simulink model "HybridShip0730"  (R2017b)
settings: Solver=ode3  StartTime=0.0  StopTime=10000  FixedStep=0.01  RelTol=1e-3
values from neighbouring files (symbols this model uses):
  Bat_Cap_Ah = Bat_Cap_kWh*1000/V_bus_nom    (= 930)    [ship_parameters0616.m]    (also in ship_parameters0616_utf8.m)
  Bat_R_int = 0.02    [ship_parameters0616.m]    (also in ship_parameters0616_utf8.m)
  Bat_SOC_init = 0.6    [ship_parameters0616.m]    (also in ship_parameters0616_utf8.m)
  C_bus = 20    [ship_parameters0616.m]    (also in ship_parameters0616_utf8.m)
  Elec_Eff = 0.92    [ship_parameters0616.m]    (also in ship_parameters0616_utf8.m)
  EMS_P_Hotel = 100    [ship_parameters0616.m]    (also in ship_parameters0616_utf8.m)
  F_env_const = 0    [ship_parameters0616.m]    (also in ship_parameters0616_utf8.m)
  Gear_Eff = 0.96    [ship_parameters0616.m]    (also in ship_parameters0616_utf8.m)
  Gear_Ratio = 6.08    [ship_parameters0616.m]    (also in ship_parameters0616_utf8.m)
  Gen_Fric_B = 0.1    [ship_parameters0616.m]    (also in ship_parameters0616_utf8.m)
  Gen_J = 50    [ship_parameters0616.m]    (also in ship_parameters0616_utf8.m)
  Gen_P_max = 500    [ship_parameters0616.m]    (also in ship_parameters0616_utf8.m)
  Gen_PI_I = 20    [ship_parameters0616.m]    (also in ship_parameters0616_utf8.m)
  Gen_PI_P = 50    [ship_parameters0616.m]    (also in ship_parameters0616_utf8.m)
  Gen_RPM_max = 1700    [ship_parameters0616.m]    (also in ship_parameters0616_utf8.m)
  Gen_RPM_nom = 1500    [ship_parameters0616.m]    (also in ship_parameters0616_utf8.m)
  Hull_K_R = P_effective_design_W / V_design_mps^3    (= 2651.6780136)    [ship_parameters0616.m]    (also in ship_parameters0616_utf8.m)
  K_Fv = (F_bollard - F_eff_design) / V_A_design^2    (= 1835.07128969)    [ship_parameters0616.m]    (also in ship_parameters0616_utf8.m)
  K_Fw = F_bollard / omega_prop_nom^2    (= 100.917597758)    [ship_parameters0616.m]    (also in ship_parameters0616_utf8.m)
  K_Qv = (Q_bollard - Q_prop_nom) / V_A_design^2    (= 212.582578785)    [ship_parameters0616.m]    (also in ship_parameters0616_utf8.m)
  K_Qw = Q_bollard / omega_prop_nom^2    (= 23.3814602154)    [ship_parameters0616.m]    (also in ship_parameters0616_utf8.m)
  Mot_PI_I = 5    [ship_parameters0616.m]    (also in ship_parameters0616_utf8.m)
  Mot_PI_P = 20    [ship_parameters0616.m]    (also in ship_parameters0616_utf8.m)
  Mot_T_max = (Mot_P_nom*1000)/(2*pi*Mot_RPM_nom/60)    (= 2228.16920329)    [ship_parameters0616.m]    (also in ship_parameters0616_utf8.m)
  Prop_J = 800    [ship_parameters0616.m]    (also in ship_parameters0616_utf8.m)
  R_tie = 0.002    [ship_parameters0616.m]    (also in ship_parameters0616_utf8.m)
  River_Current_mps = -1.0    (= -1)    [ship_parameters0616.m]    (also in ship_parameters0616_utf8.m)
  Shaft_B = 0    [ship_parameters0616.m]    (also in ship_parameters0616_utf8.m)
  Ship_Mass = 1.0e6    (= 1000000)    [ship_parameters0616.m]    (also in ship_parameters0616_utf8.m)
  V_bus_nom = 576    [ship_parameters0616.m]    (also in ship_parameters0616_utf8.m)
  wake_fraction = 0.15    [ship_parameters0616.m]    (also in ship_parameters0616_utf8.m)
libraries: simulink x6, simulink_extras x1
settings Model: Creator=Tommy  LastModifiedBy=Tommy

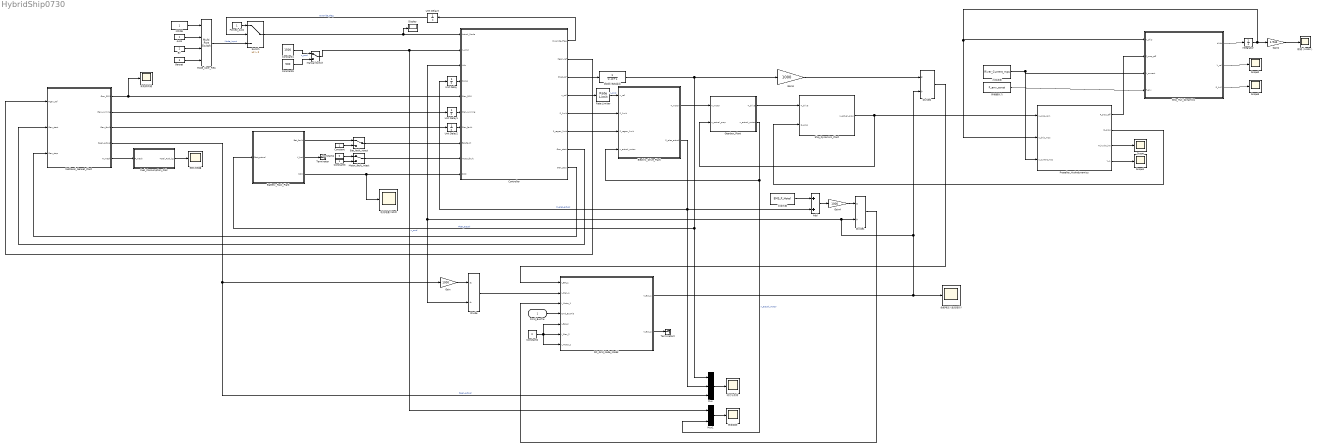
== system HybridShip0730 ==
  Cmd_BusTie : Inport
  Add : Sum
  Auto : Constant
  Bat_fault_Inject : ManualSwitch
  Battery_Pack_Plant : Subsystem
  Constant : Constant
  Constant1 : Constant  Value=1500  VectorParams1D=off  SampleTime=-1
  Constant2 : Constant  Value=0
  Constant3 : Constant
  Constant4 : Constant  Value=0
  Constant5 : Constant  Value=500  VectorParams1D=off  SampleTime=-1
  Controller : MATLAB Function  TreatAsAtomicUnit=on
  DCDC 响应延迟 : TransferFcn  Denominator=[0.1 1]
  DC_Grid_Node_Model : Subsystem
  Display : Display
  Divide : Product  Inputs=*/
  Divide1 : Product  Inputs=*/
  Divide2 : Product  Inputs=*/
  EV : Constant  Value=2
  Electric_Drive_Plant : Subsystem
  Forced_Auto : Constant
  Fuel_Consumption_Calc : Subsystem
  Gain : Gain  Gain=1000
  Gain2 : Gain  Gain=1.944
  Gain3 : Gain  Gain=1000
  Gain4 : Gain  Gain=1000
  Gearbox_Plant : Subsystem
  Genset : Constant  Value=3
  Integrator : Integrator
  MODE : Constant
  Manual Switch : ManualSwitch
  Methanol_Genset_Plant : Subsystem
  Mode_User_Req : MultiPortSwitch
  Motor_fault_Inject : ManualSwitch
  Mux : Mux  Inputs=3
  Mux1 : Mux  Inputs=2
  Propeller_Hydrodynamics : MATLAB Function  TreatAsAtomicUnit=on
  Rate Limiter : RateLimiter  RisingSlewLimit=50  FallingSlewLimit=-50  SampleTimeMode=inherited
  Scope{,1..3} (4 alike) : Scope
  Ship_Dynamics_Plant : Subsystem
  Ship_Hull_Dynamics : MATLAB Function  TreatAsAtomicUnit=on
  Switch : Switch  Criteria=u2 > Threshold
  Terminator : Terminator
  Terminator2 : Terminator
  Unit Delay{,1..3} (4 alike) : UnitDelay  SampleTime=0.1
  全船电压 (直流母排) : Scope
  动力与负荷 : Scope
  发电机转速 : Scope
  日用负载 : Constant  Value=EMS_P_Hotel
  河流流速 : Constant  Value=River_Current_mps
  燃料消耗量 : Scope
  环境额外力 : Constant  Value=F_env_const
  电池电量 (SOC) : Scope
  船速（knots） : Scope
  转速追踪 : Scope
  wires:
  Cmd_BusTie/1 -> DC_Grid_Node_Model/4(Cmd_BusTie)
  Methanol_Genset_Plant/4(Pgen_actual) -> Mux/3, Gain/1  "Pgen_actual"
  Gain/1 -> Divide/1
  Divide/1 -> DC_Grid_Node_Model/2(I_Gen_1)
  Controller/3(Pbat_ref) -> DCDC 响应延迟/1
  DCDC 响应延迟/1 -> Mux/1, Battery_Pack_Plant/1(Pbat_actual), Gain3/1  "Pbat_actual"
  Gain3/1 -> Divide2/1
  Divide2/1 -> DC_Grid_Node_Model/1(I_Bat_1)
  Electric_Drive_Plant/2(P_elec_actual) -> Add/2, Unit Delay/1, Mux/2  "P_elec_actual"
  Gain4/1 -> Divide1/1
  Divide1/1 -> DC_Grid_Node_Model/3(I_Motor_1)
  DC_Grid_Node_Model/1(V_Bus_1) -> Divide2/2, Divide/2, Controller/3(Vdc), Divide1/2, 全船电压 (直流母排)/1
  Methanol_Genset_Plant/2(Gen_running) -> Unit Delay1/1
  Battery_Pack_Plant/3(SOC) -> 电池电量 (SOC)/1, Controller/10(SOC)
  Controller/2(Pgen_ref) -> Methanol_Genset_Plant/1(Pgen_ref)
  Controller/7(Gen_start) -> Methanol_Genset_Plant/2(Gen_start)
  Controller/8(Gen_stop) -> Methanol_Genset_Plant/3(Gen_stop)
  Battery_Pack_Plant/2(V_bat) -> Terminator/1
  Battery_Pack_Plant/1(Bat_fault) -> Bat_fault_Inject/1
  DC_Grid_Node_Model/2(V_Bus_2) -> Terminator2/1
  Constant2/1 -> DC_Grid_Node_Model/7(I_Motor_2), DC_Grid_Node_Model/5(I_Bat_2), DC_Grid_Node_Model/6(I_Gen_2)
  Mux/1 -> 动力与负荷/1
  Mux1/1 -> 转速追踪/1
  Unit Delay1/1 -> Controller/6(Gen_running)
  Unit Delay/1 -> Controller/4(Pprop)
  Unit Delay2/1 -> Controller/7(Gen_fault)
  Controller/5(P_limit) -> Electric_Drive_Plant/2(P_limit)
  Controller/4(n_ref) -> Rate Limiter/1
  Electric_Drive_Plant/1(T_motor) -> Gearbox_Plant/1(T_motor)
  Gearbox_Plant/1(T_drive) -> Ship_Dynamics_Plant/1(T_drive)
  Gearbox_Plant/2(n_actual_motor) -> Mux1/2, Electric_Drive_Plant/4(n_actual_motor)  "n_actual_motor"
  Manual Switch/1 -> Mux1/1, Controller/2(n_cmd)  "n_cmd"
  Rate Limiter/1 -> Electric_Drive_Plant/1(n_ref)  "n_cmd"
  Auto/1 -> Mode_User_Req/2
  EV/1 -> Mode_User_Req/3
  Genset/1 -> Mode_User_Req/4
  MODE/1 -> Mode_User_Req/1
  Forced_Auto/1 -> Switch/1
  Mode_User_Req/1 -> Switch/3  "Mode_input"
  Switch/1 -> Controller/1(Actual_Mode), Display/1
  Controller/1(Override_Flag) -> Unit Delay3/1
  Unit Delay3/1 -> Switch/2  "Override_Flag"
  Fuel_Consumption_Calc/1(Total_Fuel_kg) -> 燃料消耗量/1
  Methanol_Genset_Plant/5(P_mech) -> Fuel_Consumption_Calc/1(P_mech)
  Bat_fault_Inject/1 -> Controller/8(Bat_fault)
  Motor_fault_Inject/1 -> Controller/9(Motor_fault)
  Constant/1 -> Bat_fault_Inject/2
  Constant3/1 -> Motor_fault_Inject/2
  Controller/6(P_regen_limit) -> Electric_Drive_Plant/3(P_regen_limit)
  Constant4/1 -> Motor_fault_Inject/1
  Methanol_Genset_Plant/3(Gen_fault) -> Unit Delay2/1
  Methanol_Genset_Plant/1(Gen_RPM) -> 发电机转速/1, Controller/5(Gen_RPM)
  Ship_Hull_Dynamics/1(dVdt) -> Integrator/1
  Integrator/1 -> Ship_Hull_Dynamics/1(V_ship), Propeller_Hydrodynamics/2(V_ship_mps), Gain2/1
  Gain2/1 -> 船速（knots）/1
  Ship_Dynamics_Plant/1(n_actual_prop) -> Propeller_Hydrodynamics/1(n_prop_rpm), Gearbox_Plant/2(n_actual_prop)
  Propeller_Hydrodynamics/2(Q_prop) -> Ship_Dynamics_Plant/2(Q_prop)
  Propeller_Hydrodynamics/1(F_prop_eff) -> Ship_Hull_Dynamics/2(F_prop_eff)
  河流流速/1 -> Ship_Hull_Dynamics/3(V_current), Propeller_Hydrodynamics/3(V_current_mps)
  环境额外力/1 -> Ship_Hull_Dynamics/4(F_env)
  Propeller_Hydrodynamics/3(P_hydro_kW) -> Scope/1
  Propeller_Hydrodynamics/4(V_A) -> Scope1/1
  Ship_Hull_Dynamics/2(V_rel) -> Scope2/1
  Ship_Hull_Dynamics/3(R_hull) -> Scope3/1
  Constant1/1 -> Manual Switch/1  "n_cmd"
  Constant5/1 -> Manual Switch/2
  Add/1 -> Gain4/1
  日用负载/1 -> Add/1

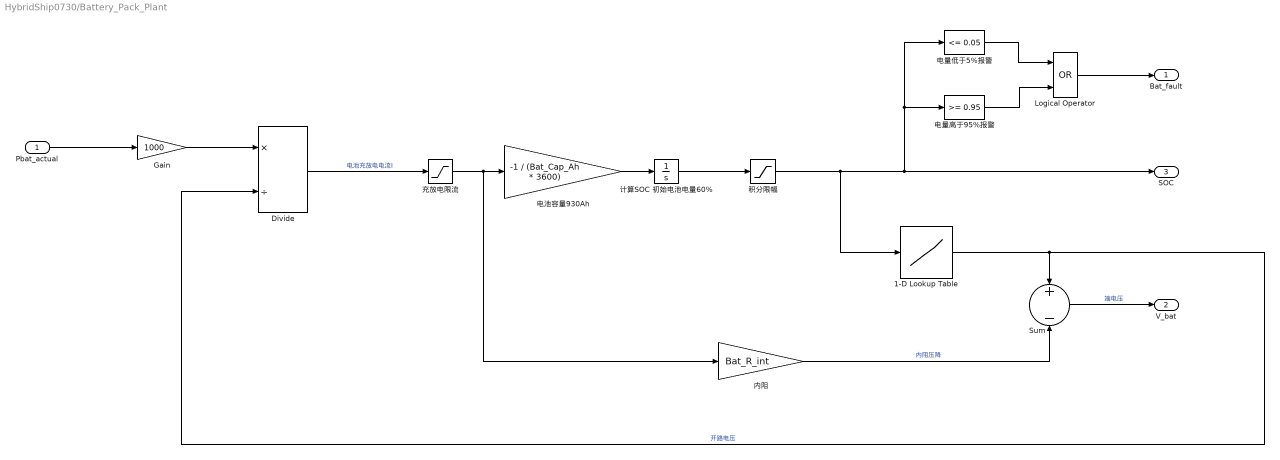
== system HybridShip0730/Battery_Pack_Plant ==
  Pbat_actual : Inport
  1-D Lookup Table : Lookup_n-D  NumberOfTableDimensions=1  BreakpointsForDimension1=[0, 0.1, 0.2, 0.5, 0.8, 0.9, 1.0]  Table=[504, 558, 576, 594, 603, 621, 657]  InternalRulePriority=Speed  RndMeth=Simplest  InputSameDT=on
  Divide : Product  Inputs=*/
  Gain : Gain  Gain=1000
  Logical Operator : Logic  Operator=OR  AllPortsSameDT=off  OutDataTypeStr=boolean
  Sum : Sum  Inputs=+-
  充放电限流 : Saturate  UpperLimit=500  LowerLimit=-500
  内阻 : Gain  Gain=Bat_R_int
  电池容量930Ah : Gain  Gain=-1 / (Bat_Cap_Ah * 3600)
  电量低于5%报警 : simulink/Logic and Bit Operations/Compare To Constant  relop=<=  const=0.05  OutDataTypeStr=boolean
  电量高于95%报警 : simulink/Logic and Bit Operations/Compare To Constant  relop=>=  const=0.95  OutDataTypeStr=boolean
  积分限幅 : Saturate  UpperLimit=1  LowerLimit=0
  计算SOC 初始电池电量60% : Integrator  InitialCondition=Bat_SOC_init
  Bat_fault : Outport
  V_bat : Outport  Port=2
  SOC : Outport  Port=3
  wires:
  Pbat_actual/1 -> Gain/1
  Gain/1 -> Divide/1
  Divide/1 -> 充放电限流/1  "电池充放电电流I"
  电池容量930Ah/1 -> 计算SOC 初始电池电量60%/1
  计算SOC 初始电池电量60%/1 -> 积分限幅/1
  积分限幅/1 -> SOC/1, 电量低于5%报警/1, 电量高于95%报警/1, 1-D Lookup Table/1
  1-D Lookup Table/1 -> Sum/1, Divide/2  "开路电压"
  内阻/1 -> Sum/2  "内阻压降"
  Sum/1 -> V_bat/1  "端电压"
  电量低于5%报警/1 -> Logical Operator/1
  电量高于95%报警/1 -> Logical Operator/2
  Logical Operator/1 -> Bat_fault/1
  充放电限流/1 -> 内阻/1, 电池容量930Ah/1

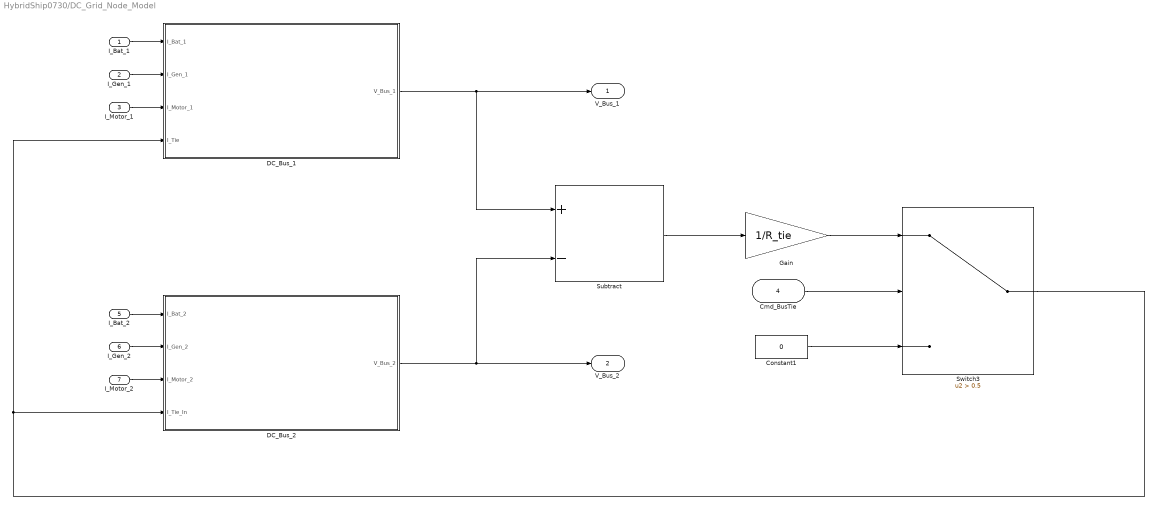
== system HybridShip0730/DC_Grid_Node_Model ==
  I_Bat_1 : Inport
  I_Gen_1 : Inport  Port=2
  I_Motor_1 : Inport  Port=3
  Cmd_BusTie : Inport  Port=4
  I_Bat_2 : Inport  Port=5
  I_Gen_2 : Inport  Port=6
  I_Motor_2 : Inport  Port=7
  Constant1 : Constant  Value=0
  DC_Bus_1 : Subsystem
  DC_Bus_2 : Subsystem
  Gain : Gain  Gain=1/R_tie
  Subtract : Sum  Inputs=+-
  Switch3 : Switch  Criteria=u2 > Threshold  Threshold=0.5
  V_Bus_1 : Outport
  V_Bus_2 : Outport  Port=2
  wires:
  I_Gen_2/1 -> DC_Bus_2/2(I_Gen_2)
  I_Gen_1/1 -> DC_Bus_1/2(I_Gen_1)
  I_Bat_2/1 -> DC_Bus_2/1(I_Bat_2)
  I_Bat_1/1 -> DC_Bus_1/1(I_Bat_1)
  I_Motor_2/1 -> DC_Bus_2/3(I_Motor_2)
  I_Motor_1/1 -> DC_Bus_1/3(I_Motor_1)
  Switch3/1 -> DC_Bus_2/4(I_Tie_In), DC_Bus_1/4(I_Tie)
  Cmd_BusTie/1 -> Switch3/2
  Constant1/1 -> Switch3/3
  DC_Bus_2/1(V_Bus_2) -> V_Bus_2/1, Subtract/2
  Subtract/1 -> Gain/1
  Gain/1 -> Switch3/1
  DC_Bus_1/1(V_Bus_1) -> V_Bus_1/1, Subtract/1

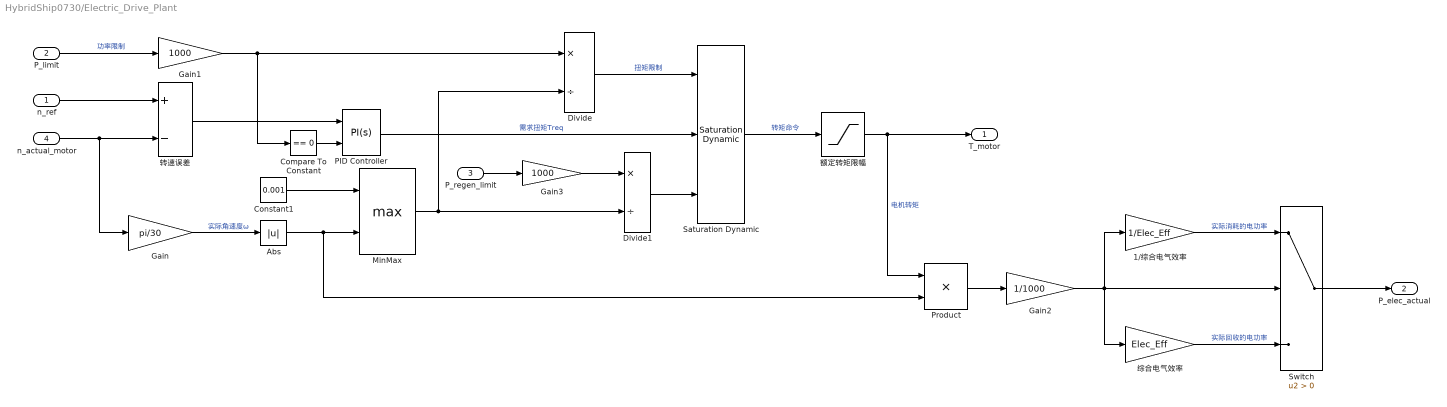
== system HybridShip0730/Electric_Drive_Plant ==
  n_ref : Inport
  P_limit : Inport  Port=2
  P_regen_limit : Inport  Port=3
  n_actual_motor : Inport  Port=4
  1/综合电气效率 : Gain  Gain=1/Elec_Eff
  Abs : Abs
  Compare To Constant : simulink/Logic and Bit Operations/Compare To Constant  relop===  const=0  OutDataTypeStr=boolean
  Constant1 : Constant  Value=0.001
  Divide : Product  Inputs=*/
  Divide1 : Product  Inputs=*/
  Gain : Gain  Gain=pi/30
  Gain1 : Gain  Gain=1000
  Gain2 : Gain  Gain=1/1000
  Gain3 : Gain  Gain=1000
  MinMax : MinMax  Function=max  Inputs=2
  PID Controller : simulink/Continuous/PID Controller  Controller=PI  TimeDomain=Continuous-time  SampleTime=-1  IntegratorMethod=Forward Euler  FilterMethod=Forward Euler  Form=Parallel  UseFilter=on  ControllerParametersSource=internal  P=Mot_PI_P  I=Mot_PI_I  D=0  N=100  InitialConditionSource=internal  InitialConditionForIntegrator=0  InitialConditionForFilter=0  ExternalReset=level  LimitOutput=on  UpperSaturationLimit=Mot_T_max  LowerSaturationLimit=-Mot_T_max  LinearizeAsGain=on  AntiWindupMode=clamping  Kb=1  TrackingMode=off  Kt=1  PParamMin=[]  PParamMax=[]  IParamMin=[]  IParamMax=[]  DParamMin=[]  DParamMax=[]  NParamMin=[]  NParamMax=[]  KbParamMin=[]  KbParamMax=[]  KtParamMin=[]  KtParamMax=[]  POutMin=[]  POutMax=[]  IOutMin=[]  IOutMax=[]  DOutMin=[]  DOutMax=[]  NOutMin=[]  NOutMax=[]  KbOutMin=[]  KbOutMax=[]  KtOutMin=[]  KtOutMax=[]  IntegratorOutMin=[]  IntegratorOutMax=[]  FilterOutMin=[]  FilterOutMax=[]  SumOutMin=[]  SumOutMax=[]  SumI1OutMin=[]  SumI1OutMax=[]  SumI2OutMin=[]  SumI2OutMax=[]  SumI3OutMin=[]  SumI3OutMax=[]  SumDOutMin=[]  SumDOutMax=[]  SaturationOutMin=[]  SaturationOutMax=[]  IntegratorContinuousStateAttributes=''  IntegratorStateMustResolveToSignalObject=off  IntegratorRTWStateStorageClass=Auto  FilterContinuousStateAttributes=''  FilterStateMustResolveToSignalObject=off  FilterRTWStateStorageClass=Auto  DifferentiatorICPrevScaledInput=0  DifferentiatorOutMin=[]  DifferentiatorOutMax=[]  InitialConditionSetting=State (most efficient)  FilterDiffOutCoefMin=[]  FilterDiffOutCoefMax=[]  SumDenOutMin=[]  SumDenOutMax=[]  SumNumOutMin=[]  SumNumOutMax=[]  ReciprocalOutMin=[]  ReciprocalOutMax=[]  DivideOutMin=[]  DivideOutMax=[]  TunerSelectOption=Transfer Function Based (PID Tuner App)
  Product : Product
  Saturation Dynamic : simulink/Discontinuities/Saturation Dynamic  OutMin=[]  OutMax=[]  OutDataTypeStr=Inherit: Same as second input  OutDataType=fixdt(1, 16)  OutScaling=2^-10  DoSatur=off
  Switch : Switch  Criteria=u2 > Threshold
  综合电气效率 : Gain  Gain=Elec_Eff
  转速误差 : Sum  Inputs=+-
  额定转矩限幅 : Saturate  UpperLimit=Mot_T_max  LowerLimit=-Mot_T_max
  T_motor : Outport
  P_elec_actual : Outport  Port=2
  wires:
  n_ref/1 -> 转速误差/1
  n_actual_motor/1 -> 转速误差/2, Gain/1
  转速误差/1 -> PID Controller/1
  PID Controller/1 -> Saturation Dynamic/2  "需求扭矩Treq"
  Gain1/1 -> Divide/1, Compare To Constant/1
  P_limit/1 -> Gain1/1  "功率限制"
  Gain/1 -> Abs/1  "实际角速度ω"
  MinMax/1 -> Divide/2, Divide1/2
  Divide/1 -> Saturation Dynamic/1  "扭矩限制"
  Constant1/1 -> MinMax/1
  Gain2/1 -> 综合电气效率/1, 1/综合电气效率/1, Switch/2
  Product/1 -> Gain2/1
  Switch/1 -> P_elec_actual/1
  Saturation Dynamic/1 -> 额定转矩限幅/1  "转矩命令"
  额定转矩限幅/1 -> Product/1, T_motor/1  "电机转矩"
  P_regen_limit/1 -> Gain3/1
  Gain3/1 -> Divide1/1
  Divide1/1 -> Saturation Dynamic/3
  Abs/1 -> MinMax/2, Product/2
  1/综合电气效率/1 -> Switch/1  "实际消耗的电功率"
  综合电气效率/1 -> Switch/3  "实际回收的电功率"
  Compare To Constant/1 -> PID Controller/2

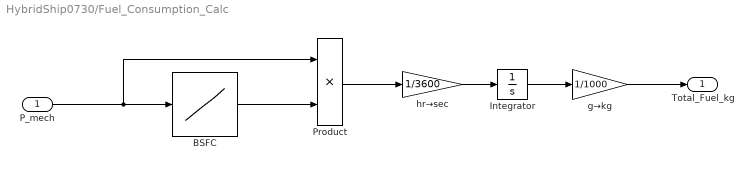
== system HybridShip0730/Fuel_Consumption_Calc ==
  P_mech : Inport
  BSFC : Lookup_n-D  NumberOfTableDimensions=1  BreakpointsForDimension1=[0, 50, 100, 200, 300, 400, 500]  Table=[1200, 700, 550, 480, 450, 430, 460]  InternalRulePriority=Speed  RndMeth=Simplest  InputSameDT=on
  Integrator : Integrator
  Product : Product
  g→kg : Gain  Gain=1/1000
  hr→sec : Gain  Gain=1/3600
  Total_Fuel_kg : Outport
  wires:
  P_mech/1 -> Product/1, BSFC/1
  BSFC/1 -> Product/2
  Product/1 -> hr→sec/1
  hr→sec/1 -> Integrator/1
  Integrator/1 -> g→kg/1
  g→kg/1 -> Total_Fuel_kg/1

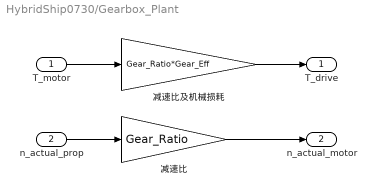
== system HybridShip0730/Gearbox_Plant ==
  T_motor : Inport
  n_actual_prop : Inport  Port=2
  减速比 : Gain  Gain=Gear_Ratio
  减速比及机械损耗 : Gain  Gain=Gear_Ratio*Gear_Eff
  T_drive : Outport
  n_actual_motor : Outport  Port=2
  wires:
  T_motor/1 -> 减速比及机械损耗/1
  减速比及机械损耗/1 -> T_drive/1
  n_actual_prop/1 -> 减速比/1
  减速比/1 -> n_actual_motor/1

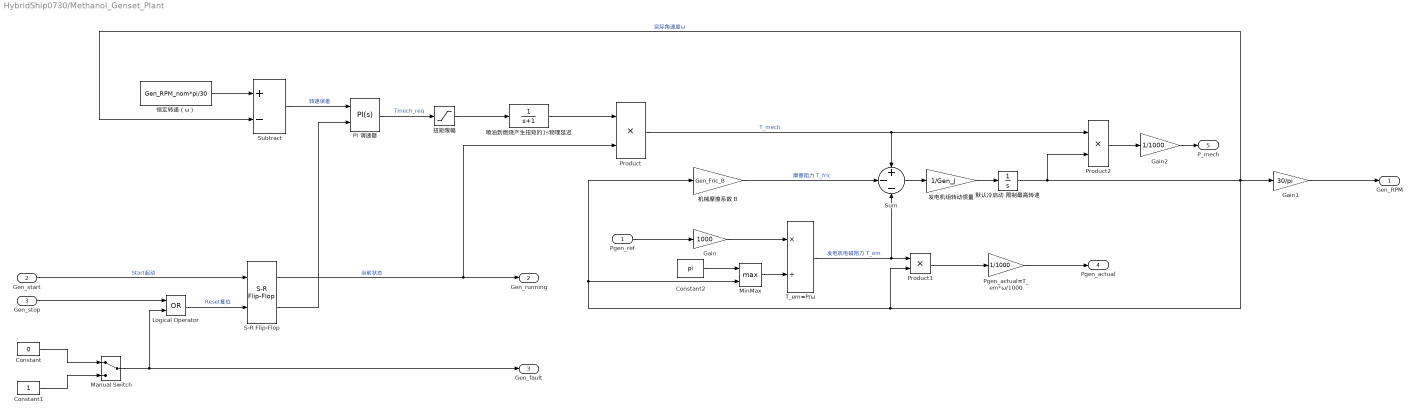
== system HybridShip0730/Methanol_Genset_Plant ==
  Pgen_ref : Inport
  Gen_start : Inport  Port=2
  Gen_stop : Inport  Port=3
  Constant : Constant  Value=0
  Constant1 : Constant
  Constant2 : Constant  Value=pi
  Gain : Gain  Gain=1000
  Gain1 : Gain  Gain=30/pi
  Gain2 : Gain  Gain=1/1000
  Logical Operator : Logic  Operator=OR  AllPortsSameDT=off  OutDataTypeStr=boolean
  Manual Switch : ManualSwitch
  MinMax : MinMax  Function=max  Inputs=2
  PI 调速器 : simulink/Continuous/PID Controller  Controller=PI  TimeDomain=Continuous-time  SampleTime=-1  IntegratorMethod=Forward Euler  FilterMethod=Forward Euler  Form=Parallel  UseFilter=on  ControllerParametersSource=internal  P=Gen_PI_P  I=Gen_PI_I  D=0  N=100  InitialConditionSource=internal  InitialConditionForIntegrator=0  InitialConditionForFilter=0  ExternalReset=level  LimitOutput=off  UpperSaturationLimit=inf  LowerSaturationLimit=-inf  LinearizeAsGain=on  AntiWindupMode=none  Kb=1  TrackingMode=off  Kt=1  PParamMin=[]  PParamMax=[]  IParamMin=[]  IParamMax=[]  DParamMin=[]  DParamMax=[]  NParamMin=[]  NParamMax=[]  KbParamMin=[]  KbParamMax=[]  KtParamMin=[]  KtParamMax=[]  POutMin=[]  POutMax=[]  IOutMin=[]  IOutMax=[]  DOutMin=[]  DOutMax=[]  NOutMin=[]  NOutMax=[]  KbOutMin=[]  KbOutMax=[]  KtOutMin=[]  KtOutMax=[]  IntegratorOutMin=[]  IntegratorOutMax=[]  FilterOutMin=[]  FilterOutMax=[]  SumOutMin=[]  SumOutMax=[]  SumI1OutMin=[]  SumI1OutMax=[]  SumI2OutMin=[]  SumI2OutMax=[]  SumI3OutMin=[]  SumI3OutMax=[]  SumDOutMin=[]  SumDOutMax=[]  SaturationOutMin=[]  SaturationOutMax=[]  IntegratorContinuousStateAttributes=''  IntegratorStateMustResolveToSignalObject=off  IntegratorRTWStateStorageClass=Auto  FilterContinuousStateAttributes=''  FilterStateMustResolveToSignalObject=off  FilterRTWStateStorageClass=Auto  DifferentiatorICPrevScaledInput=0  DifferentiatorOutMin=[]  DifferentiatorOutMax=[]  InitialConditionSetting=State (most efficient)  FilterDiffOutCoefMin=[]  FilterDiffOutCoefMax=[]  SumDenOutMin=[]  SumDenOutMax=[]  SumNumOutMin=[]  SumNumOutMax=[]  ReciprocalOutMin=[]  ReciprocalOutMax=[]  DivideOutMin=[]  DivideOutMax=[]  TunerSelectOption=Transfer Function Based (PID Tuner App)
  Pgen_actual=T_em*ω/1000 : Gain  Gain=1/1000
  Product : Product
  Product1 : Product
  Product2 : Product
  S-R Flip-Flop : simulink_extras/Flip Flops/S-R Flip-Flop  initial_condition=0
  Subtract : Sum  Inputs=+-
  Sum : Sum  Inputs=+--
  T_em=P/ω : Product  Inputs=*/
  发电机组转动惯量 : Gain  Gain=1/Gen_J
  喷油到燃烧产生扭矩的1s物理延迟 : TransferFcn  Denominator=[1 1]
  恒定转速（ω） : Constant  Value=Gen_RPM_nom*pi/30
  扭矩限幅 : Saturate  UpperLimit=30000*Gen_P_max/(Gen_RPM_nom*pi)  LowerLimit=0
  机械摩擦系数 B : Gain  Gain=Gen_Fric_B
  默认冷启动 限制最高转速 : Integrator  LimitOutput=on  UpperSaturationLimit=Gen_RPM_max*pi/30  LowerSaturationLimit=0
  Gen_RPM : Outport
  Gen_running : Outport  Port=2
  Gen_fault : Outport  Port=3
  Pgen_actual : Outport  Port=4
  P_mech : Outport  Port=5
  wires:
  Gen_start/1 -> S-R Flip-Flop/1  "Start起动"
  Gen_stop/1 -> Logical Operator/1
  Constant/1 -> Manual Switch/1
  Constant1/1 -> Manual Switch/2
  Manual Switch/1 -> Gen_fault/1, Logical Operator/2
  Logical Operator/1 -> S-R Flip-Flop/2  "Reset复位"
  S-R Flip-Flop/1 -> Gen_running/1, Product/2  "当前状态"
  S-R Flip-Flop/2 -> PI 调速器/2
  Pgen_ref/1 -> Gain/1
  Constant2/1 -> MinMax/1
  Gain/1 -> T_em=P/ω/1
  恒定转速（ω）/1 -> Subtract/1
  Subtract/1 -> PI 调速器/1  "转速误差"
  PI 调速器/1 -> 扭矩限幅/1  "Tmech_req"
  扭矩限幅/1 -> 喷油到燃烧产生扭矩的1s物理延迟/1
  喷油到燃烧产生扭矩的1s物理延迟/1 -> Product/1
  Product/1 -> Sum/1, Product2/1  "T_mech"
  T_em=P/ω/1 -> Sum/3, Product1/1  "发电机电磁阻力 T_em"
  Sum/1 -> 发电机组转动惯量/1
  发电机组转动惯量/1 -> 默认冷启动 限制最高转速/1
  默认冷启动 限制最高转速/1 -> Subtract/2, Gain1/1, MinMax/2, 机械摩擦系数 B/1, Product1/2, Product2/2  "实际角速度ω"
  MinMax/1 -> T_em=P/ω/2
  Gain1/1 -> Gen_RPM/1
  Product1/1 -> Pgen_actual=T_em*ω/1000/1
  Pgen_actual=T_em*ω/1000/1 -> Pgen_actual/1
  机械摩擦系数 B/1 -> Sum/2  "摩擦阻力 T_fric"
  Product2/1 -> Gain2/1
  Gain2/1 -> P_mech/1

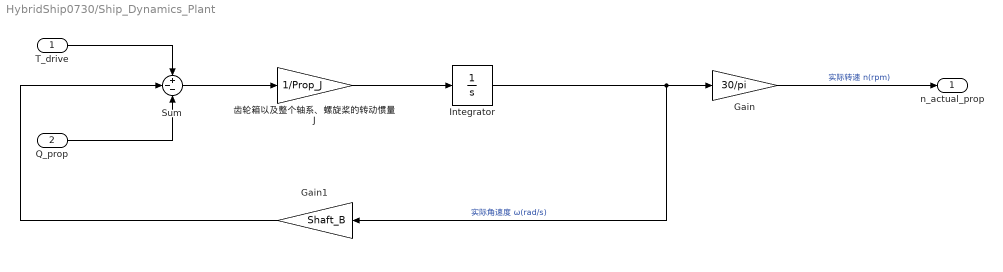
== system HybridShip0730/Ship_Dynamics_Plant ==
  T_drive : Inport
  Q_prop : Inport  Port=2
  Gain : Gain  Gain=30/pi
  Gain1 : Gain  Gain=Shaft_B
  Integrator : Integrator
  Sum : Sum  Inputs=+--
  齿轮箱以及整个轴系、螺旋桨的转动惯量 J : Gain  Gain=1/Prop_J
  n_actual_prop : Outport
  wires:
  T_drive/1 -> Sum/1
  Q_prop/1 -> Sum/3
  Sum/1 -> 齿轮箱以及整个轴系、螺旋桨的转动惯量 J/1
  齿轮箱以及整个轴系、螺旋桨的转动惯量 J/1 -> Integrator/1
  Integrator/1 -> Gain1/1, Gain/1  "实际角速度 ω(rad/s)"
  Gain/1 -> n_actual_prop/1  "实际转速 n(rpm)"
  Gain1/1 -> Sum/2

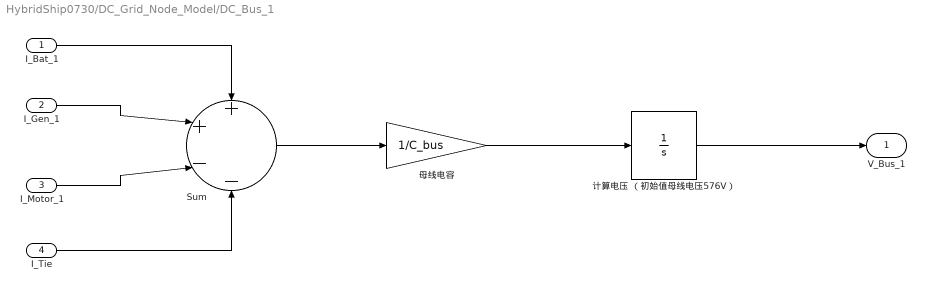
== system HybridShip0730/DC_Grid_Node_Model/DC_Bus_1 ==
  I_Bat_1 : Inport
  I_Gen_1 : Inport  Port=2
  I_Motor_1 : Inport  Port=3
  I_Tie : Inport  Port=4
  Sum : Sum  Inputs=++--
  母线电容 : Gain  Gain=1/C_bus
  计算电压 （初始值母线电压576V） : Integrator  InitialCondition=V_bus_nom
  V_Bus_1 : Outport
  wires:
  母线电容/1 -> 计算电压 （初始值母线电压576V）/1
  Sum/1 -> 母线电容/1
  I_Gen_1/1 -> Sum/2
  计算电压 （初始值母线电压576V）/1 -> V_Bus_1/1
  I_Tie/1 -> Sum/4
  I_Motor_1/1 -> Sum/3
  I_Bat_1/1 -> Sum/1

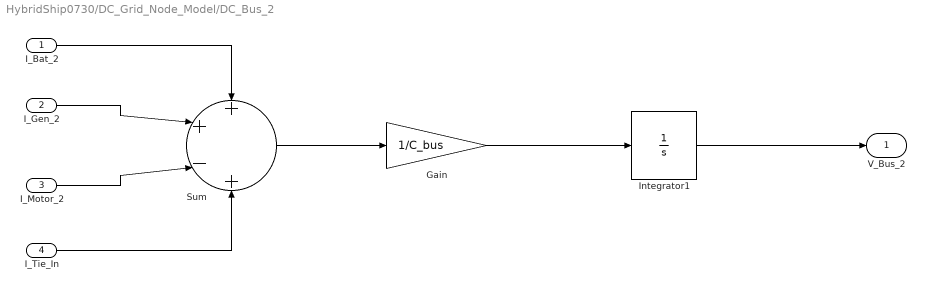
== system HybridShip0730/DC_Grid_Node_Model/DC_Bus_2 ==
  I_Bat_2 : Inport
  I_Gen_2 : Inport  Port=2
  I_Motor_2 : Inport  Port=3
  I_Tie_In : Inport  Port=4
  Gain : Gain  Gain=1/C_bus
  Integrator1 : Integrator  InitialCondition=576
  Sum : Sum  Inputs=++-+
  V_Bus_2 : Outport
  wires:
  Gain/1 -> Integrator1/1
  Sum/1 -> Gain/1
  I_Gen_2/1 -> Sum/2
  Integrator1/1 -> V_Bus_2/1
  I_Tie_In/1 -> Sum/4
  I_Motor_2/1 -> Sum/3
  I_Bat_2/1 -> Sum/1

== matlab function HybridShip0730/Ship_Hull_Dynamics ==
  data: V_ship input; dVdt output; F_prop_eff input; V_current input; F_env input; V_rel output; R_hull output; Hull_K_R parameter double size=[1 1]; Ship_Mass parameter double size=[1 1]
function [dVdt, V_rel, R_hull] = HullLongitudinalDynamics(V_ship, F_prop_eff, V_current, F_env, Hull_K_R, Ship_Mass)
% 船体纵向动力学
%
% 输入：
% V_ship      : 船舶对地速度 [m/s]
% F_prop_eff  : 螺旋桨作用到船体上的有效推力 [N]
% V_current   : 河流流速 [m/s]
% F_env       : 额外环境力 [N]
%
% 输出：
% dVdt        : 船舶对地加速度 [m/s^2]
% V_rel       : 船舶相对水速度 [m/s]
% R_hull      : 船体阻力 [N]

% 船舶相对水速度
% 船前进为正，逆流时 V_current < 0
V_rel = V_ship - V_current;

% 船体阻力，方向永远与相对水运动方向相反
R_hull = Hull_K_R * V_rel * abs(V_rel);

% 纵向运动方程
% M * dV/dt = F_prop_eff - R_hull + F_env
dVdt = (F_prop_eff - R_hull + F_env) / Ship_Mass;
end

== matlab function HybridShip0730/Controller ==
  settings: updateMethod=DISCRETE  sampleTime=0.1
  data: Actual_Mode input; n_cmd input; Override_Flag output; Vdc input; Pprop input; Gen_RPM input; Gen_running input; Gen_fault input; Bat_fault input; Motor_fault input; SOC input; Pgen_ref output; Pbat_ref output; n_ref output; P_limit output; P_regen_limit output; Gen_start output; Gen_stop output
function [Override_Flag, Pgen_ref, Pbat_ref, n_ref, P_limit, P_regen_limit, Gen_start, Gen_stop] = EMS_Controller(Actual_Mode, n_cmd, Vdc, Pprop, Gen_RPM, Gen_running, Gen_fault, Bat_fault, Motor_fault, SOC)

    % ================= 1. 参数标定 =================
    Vdc_nom = 576;              % 额定直流母线电压 [V]
    Vdc_low_cut = 500;          % 严重欠压保护阈值 [V]

    Vdc_regen_derate_start = 590;   % 回馈开始降额电压 [V]
    Vdc_regen_cut = 600;            % 回馈完全禁止电压 [V]

    P_gen_opt = 400;            % 发电机经济运行功率 [kW]
    P_gen_max = 500;            % 发电机最大功率 [kW]

    P_prop_max = 350;           % 推进电机正向最大电功率 [kW]
    P_bat_discharge_max = 500;  % 电池最大放电功率 [kW]
    P_bat_charge_max = 500;     % 电池最大充电功率 [kW]

    SOC_START = 0.25;           % 自动模式下低于该 SOC 启动发电机
    SOC_STOP  = 0.85;           % 自动模式下高于该 SOC 且负载较低时停发电机

    SOC_FORCE_EV_STOP = 0.20;   % 纯电模式低电量保护阈值
    SOC_REGEN_DERATE = 0.90;    % 高 SOC 回馈降额起点
    SOC_REGEN_STOP   = 0.95;    % 高 SOC 回馈完全禁止点

    dt = 0.1;                   % EMS 采样时间 [s]
    Ramp_Rate = 20;             % 发电机功率爬坡率 [kW/s]

    K_droop_bat = 2;            % 电池稳压下垂系数 [kW/V]
    K_droop_gen = 5;            % 电池故障时发电机稳压下垂系数 [kW/V]

    P_regen_deadband = 2;       % 判断回馈的小死区 [kW]
    Gen_warmup_rpm = 1450;      % 发电机未达到该转速前不加载 [rpm]

    persistent Pgen_last over_flag
    if isempty(Pgen_last)
        Pgen_last = 0;
        over_flag = 0;
    end

    % Pprop 的符号约定：
    % Pprop > 0 : 推进电机从直流母线取电，推进消耗功率
    % Pprop < 0 : 推进电机向直流母线回馈，制动发电
    Pprop_for_gen = max(Pprop, 0);


    % ================= 2. 越权状态机 =================
    if over_flag == 0
        if (Actual_Mode == 2) && (SOC <= SOC_FORCE_EV_STOP)
            % 纯电模式低电量保护
            over_flag = 1;

        elseif (Actual_Mode == 3) && (SOC >= SOC_REGEN_STOP) && (Pprop_for_gen < 50)
            % 甲醇模式下电池过高，且推进负载很低，允许退出甲醇强制模式
            over_flag = 1;

        elseif Gen_fault && (Actual_Mode == 3)
            % 发电机故障，强制退出甲醇模式
            over_flag = 1;

        elseif Bat_fault && (Actual_Mode == 2)
            % 电池故障，强制退出纯电模式
            over_flag = 1;
        end
    else
        if (SOC > 0.25) && (SOC < 0.90) && (~Gen_fault) && (~Bat_fault)
            % 故障/保护条件解除，归还控制权
            over_flag = 0;
        end
    end

    Override_Flag = over_flag;


    % ================= 3. 发电机启停与目标功率 =================
    Gen_start = false;
    Gen_stop = false;
    Pgen_target = 0;

    if Gen_fault && Bat_fault
        % 发电机和电池都故障：无法供能
        Pgen_target = 0;
        if Gen_running
            Gen_stop = true;
        end

    elseif Bat_fault
        % 电池故障：发电机必须接管正向负载
        if ~Gen_running
            Gen_start = true;
        end

        % 回馈功率不能送入电池，因此发电机只跟随正向推进负载
        Pgen_target = Pprop_for_gen + K_droop_gen * (Vdc_nom - Vdc);
        Pgen_target = min(max(Pgen_target, 0), P_gen_max);

    elseif Gen_fault
        % 发电机故障：目标功率归零，靠电池
        Pgen_target = 0;
        if Gen_running
            Gen_stop = true;
        end

    else
        % -------- 正常情况下，优先处理推进回馈 --------
        if Pprop < -P_regen_deadband
            % 推进电机正在回馈，发电机不应继续主动发电
            Pgen_target = 0;

            if Gen_running
                Gen_stop = true;
            end

        else
            % -------- 非回馈工况，按模式处理 --------
            if Actual_Mode == 1
                % 自动模式
                if ~Gen_running && ((SOC < SOC_START) || (Pprop_for_gen > 300))
                    Gen_start = true;
                end

                if Gen_running && (SOC > SOC_STOP) && (Pprop_for_gen < 100)
                    Gen_stop = true;
                end

                if Gen_running
                    if Pprop_for_gen > P_gen_max
                        Pgen_target = P_gen_max;

                    elseif SOC > 0.80
                        % SOC 较高时，发电机只跟随当前负载，不额外充电
                        Pgen_target = min(Pprop_for_gen, P_gen_max);

                    else
                        % SOC 不高时，让发电机运行在较经济功率附近
                        Pgen_target = P_gen_opt;
                    end
                else
                    Pgen_target = 0;
                end

            elseif Actual_Mode == 2
                % 纯电模式
                if Gen_running
                    Gen_stop = true;
                end
                Pgen_target = 0;

            elseif Actual_Mode == 3
                % 甲醇发电机模式
                if ~Gen_running
                    Gen_start = true;
                end

                Pgen_target = P_gen_opt;

                if Pprop_for_gen > P_gen_max
                    Pgen_target = P_gen_max;

                elseif SOC > 0.90
                    % SOC 很高时，不再让发电机额外给电池充电
                    Pgen_target = min(Pprop_for_gen, P_gen_max);
                end

            else
                % 未知模式，降级为自动模式的保守策略
                if ~Gen_running && ((SOC < SOC_START) || (Pprop_for_gen > 300))
                    Gen_start = true;
                end

                if Gen_running
                    Pgen_target = min(max(Pprop_for_gen, 0), P_gen_max);
                else
                    Pgen_target = 0;
                end
            end
        end
    end

    % 发电机暖机保护：转速未建立前不加载
    if Gen_running && (Gen_RPM < Gen_warmup_rpm)
        Pgen_target = 0;
    end

    % 发电机功率爬坡限制
    dP = Pgen_target - Pgen_last;
    max_dP = Ramp_Rate * dt;

    if dP > max_dP
        Pgen_ref = Pgen_last + max_dP;
    elseif dP < -max_dP
        Pgen_ref = Pgen_last - max_dP;
    else
        Pgen_ref = Pgen_target;
    end

    if Pgen_ref < 0.001
        Pgen_ref = 0;
    end

    Pgen_last = Pgen_ref;


    % ================= 4. 电池充放电能力限制 =================
    if Bat_fault
        P_bat_discharge_allow = 0;
        P_bat_charge_allow = 0;
    else
        P_bat_discharge_allow = P_bat_discharge_max;

        % 回馈/充电降额
        if (SOC >= SOC_REGEN_STOP) || (Vdc >= Vdc_regen_cut)
            P_bat_charge_allow = 0;
        else
            soc_scale = 1;
            if SOC > SOC_REGEN_DERATE
                soc_scale = (SOC_REGEN_STOP - SOC) / (SOC_REGEN_STOP - SOC_REGEN_DERATE);
                soc_scale = min(max(soc_scale, 0), 1);
            end

            vdc_scale = 1;
            if Vdc > Vdc_regen_derate_start
                vdc_scale = (Vdc_regen_cut - Vdc) / (Vdc_regen_cut - Vdc_regen_derate_start);
                vdc_scale = min(max(vdc_scale, 0), 1);
            end

            charge_scale = min(soc_scale, vdc_scale);
            P_bat_charge_allow = P_bat_charge_max * charge_scale;
        end
    end


    % ================= 5. 电池功率指令与母线稳压 =================
    if Bat_fault
        Pbat_ref = 0;
    else
        % 正值：电池放电
        % 负值：电池充电
        Pbat_req = Pprop - Pgen_ref;

        % 母线电压低：Vdc_nom - Vdc 为正，电池多放电
        % 母线电压高：Vdc_nom - Vdc 为负，电池少放电或吸收功率
        Pbat_ref = Pbat_req + K_droop_bat * (Vdc_nom - Vdc);

        % 放电上限
        if Pbat_ref > P_bat_discharge_allow
            Pbat_ref = P_bat_discharge_allow;
        end

        % 充电/回馈吸收上限
        if Pbat_ref < -P_bat_charge_allow
            Pbat_ref = -P_bat_charge_allow;
        end
    end


    % ================= 6. 推进控制与正向功率限制 =================
    n_ref = n_cmd;

    if Motor_fault
        % 推进电机故障：切断推进与回馈
        P_limit = 0;
        n_ref = 0;

    elseif Gen_fault && (SOC < 0.15)
        % 发电机故障且电池严重低电量：失去动力来源
        P_limit = 0;
        n_ref = 0;

    elseif Gen_fault
        % 发电机故障但电池还有电：限功率航行
        P_limit = 100;

    elseif Vdc < Vdc_low_cut
        % 严重欠压：禁止正向牵引功率
        % 注意：如果回馈仍被允许，负转矩仍可用于抬升母线
        P_limit = 0;

    else
        P_limit = P_prop_max;
    end


    % ================= 7. 反向回馈功率限制 =================
    if Motor_fault || Bat_fault
        % 电机故障或电池故障：禁止回馈
        P_regen_limit = 0;

    elseif (Vdc >= Vdc_regen_cut) || (SOC >= SOC_REGEN_STOP)
        % 母线过压或电池满电：禁止回馈
        P_regen_limit = 0;

    else
        % 回馈功率不能超过推进系统能力，也不能超过电池当前可吸收能力
        P_regen_allow = min(P_prop_max, P_bat_charge_allow);

        % 输出为负值，供 Electric_Drive_Plant 的 Dynamic Saturation 下限使用
        P_regen_limit = -P_regen_allow;
    end
end

== matlab function HybridShip0730/Propeller_Hydrodynamics ==
  data: n_prop_rpm input; F_prop_eff output; V_ship_mps input; V_current_mps input; Q_prop output; P_hydro_kW output; V_A output; wake_fraction parameter double size=[1 1]; K_Fw parameter double size=[1 1]; K_Fv parameter double size=[1 1]; K_Qw parameter double size=[1 1]; K_Qv parameter double size=[1 1]
function [F_prop_eff, Q_prop, P_hydro_kW, V_A] = PropellerHydroSimple(n_prop_rpm, V_ship_mps, V_current_mps, wake_fraction, K_Fw, K_Fv, K_Qw, K_Qv)
% 简化螺旋桨水动力模型
%
% 输入：
% n_prop_rpm     : 螺旋桨转速 [rpm]
% V_ship_mps     : 船舶对地速度 [m/s]
% V_current_mps  : 河流流速 [m/s]
%
% 输出：
% F_prop_eff     : 螺旋桨有效推力 [N]
% Q_prop         : 螺旋桨水动力扭矩 [Nm]
% P_hydro_kW     : 螺旋桨吸收的轴功率 [kW]
% V_A            : 螺旋桨进速 [m/s]

% rpm -> rad/s
omega = n_prop_rpm * pi / 30;

% 船舶相对水速度
V_rel = V_ship_mps - V_current_mps;

% 螺旋桨处进速
V_A = (1 - wake_fraction) * V_rel;

% 有效推力模型
% 正值：向前推进
% 负值：螺旋桨变成阻力，拖慢船舶
F_prop_eff = K_Fw * omega * abs(omega) - K_Fv * V_A * abs(V_A);

% 水动力扭矩模型
% 正值：水动力扭矩阻碍螺旋桨正转
% 负值：水流推动螺旋桨正转，也就是 windmilling / 回拖
Q_prop = K_Qw * omega * abs(omega) - K_Qv * V_A * abs(V_A);

% 螺旋桨轴功率
% 正值：螺旋桨从轴系吸收功率
% 负值：水流给轴系输入功率
P_hydro_kW = Q_prop * omega / 1000;
end
